simulink model "Lab0_actual"  (R2024b)
settings: Solver=ode5  StartTime=0.0  StopTime=20  FixedStep=1e-03  RelTol=1e-3
undefined symbols (not defined in the file): degs2rpm, delta_i, DiscIntNeverNeededParam, gbox, Kd, Ki, Kp, mot, National_Instruments, PCI, sens, TL, wc, wc2
libraries: simulink x9, sldrtlib x3
settings Model: SimulationMode=external  ExtModeTrigDuration=45001  Creator=lenovo  LastModifiedBy=aboulenien
settings DataIOCC: ReturnWorkspaceOutputs=off
settings HardwareCC: ProdBitPerLong=64  ProdHWDeviceType=Intel->x86-64 (Linux 64)
settings RTWCC: Description=Simulink Desktop Real-Time  SystemTargetFile=sldrt.tlc  TemplateMakefile=sldrt.tmf  RTWCompilerOptimization=on
settings CodeAppCC: MaxIdLength=95
settings SimulinkDesktopRealTimeCC: TargetLibSuffix=_sldrt.a  TargetPreCompLibLocation=C:\Program Files\MATLAB\R2024b\toolbox\sldrt\lib\win64  ParMdlRefBuildCompliant=on

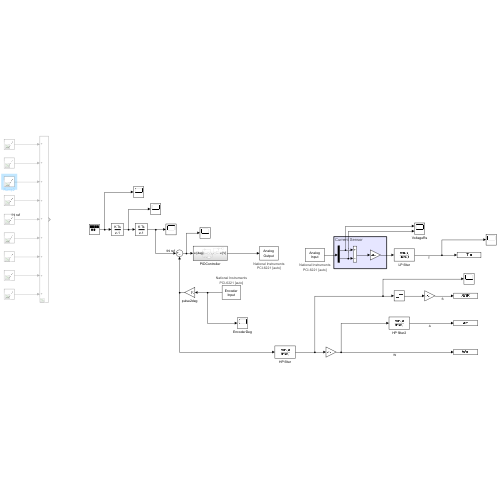
[thumbnail: Simulink's stored preview of the top-level diagram]
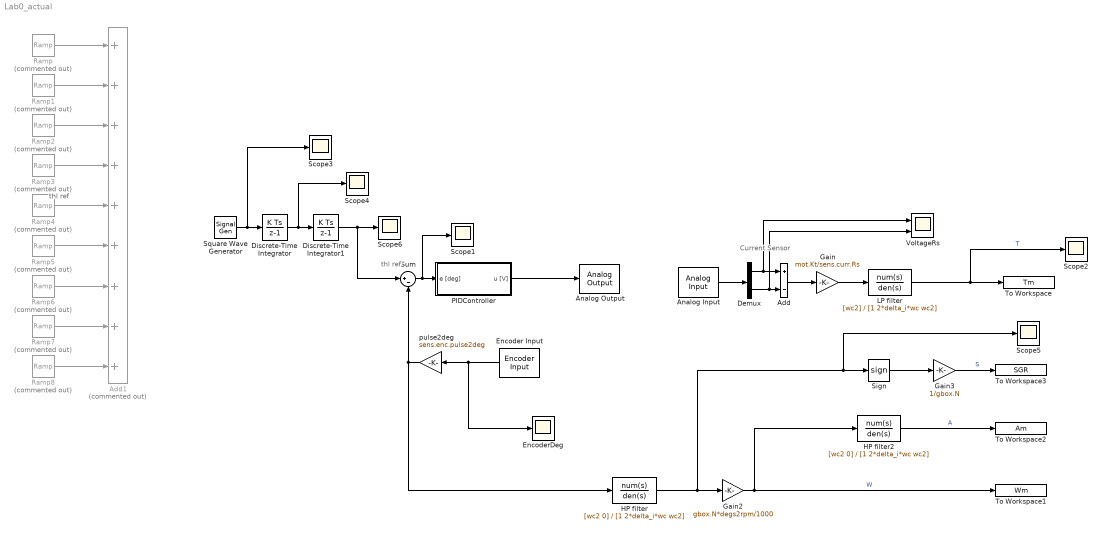
== system Lab0_actual ==
  note: Current Sensor
  note: thl ref
  note: thl ref
  Add : Sum  Inputs=+-
  Add1 : Sum  Commented=on  Inputs=+++++++++
  Analog Input : sldrtlib/Analog Input  SampleTime=-1  MaxMissedTicks=10  ShowMissedTicks=off  YieldWhenWaiting=off  DrvName=National_Instruments/PCI-6221  DrvAddress=4294967295  DrvOptions=[0 0 0 2 0]  Channels=[1,2]  RangeMode=1  VoltRange=1  DataType=1
      settings: AttributesFormatString=National Instruments\nPCI-6221 [auto]
  Analog Output : sldrtlib/Analog Output  SampleTime=-1  MaxMissedTicks=10  ShowMissedTicks=off  YieldWhenWaiting=off  DrvName=National_Instruments/PCI-6221  DrvAddress=4294967295  DrvOptions=[0 0 0 2 0]  Channels=1  RangeMode=1  VoltRange=1  InitialValue=0  FinalValue=0
      settings: AttributesFormatString=National Instruments\nPCI-6221 [auto]
  Demux : Demux  Outputs=2
  Discrete-Time Integrator : DiscreteIntegrator  SampleTime=-1  ICPrevOutput=DiscIntNeverNeededParam  ICPrevScaledInput=DiscIntNeverNeededParam
  Discrete-Time Integrator1 : DiscreteIntegrator  SampleTime=-1  ICPrevOutput=DiscIntNeverNeededParam  ICPrevScaledInput=DiscIntNeverNeededParam
  Encoder Input : sldrtlib/Encoder Input  SampleTime=-1  MaxMissedTicks=10  ShowMissedTicks=off  YieldWhenWaiting=off  DrvName=National_Instruments/PCI-6221  DrvAddress=4294967295  DrvOptions=[0 0 0 2 0]  Channels=1  QuadMode=3  IndexPulse=1  InputFilter=Inf  DataType=1
      settings: AttributesFormatString=National Instruments\nPCI-6221 [auto]
  EncoderDeg : Scope
  Gain : Gain  Gain=mot.Kt/sens.curr.Rs
  Gain2 : Gain  Gain=gbox.N*degs2rpm/1000
  Gain3 : Gain  Gain=1/gbox.N
  HP filter : TransferFcn  Numerator=[wc2 0]  Denominator=[1 2*delta_i*wc wc2]
  HP filter2 : TransferFcn  Numerator=[wc2 0]  Denominator=[1 2*delta_i*wc wc2]
  LP filter : TransferFcn  Numerator=[wc2]  Denominator=[1 2*delta_i*wc wc2]
  PIDController : Subsystem
  Ramp : simulink/Sources/Ramp  Commented=on  slope=300  start=0  InitialOutput=0
  Ramp1 : simulink/Sources/Ramp  Commented=on  slope=300  start=5  InitialOutput=0
  Ramp2 : simulink/Sources/Ramp  Commented=on  slope=300  start=10  InitialOutput=0
  Ramp3 : simulink/Sources/Ramp  Commented=on  slope=300  start=15  InitialOutput=0
  Ramp4 : simulink/Sources/Ramp  Commented=on  slope=300  start=20  InitialOutput=0
  Ramp5 : simulink/Sources/Ramp  Commented=on  slope=300  start=25  InitialOutput=0
  Ramp6 : simulink/Sources/Ramp  Commented=on  slope=300  start=30  InitialOutput=0
  Ramp7 : simulink/Sources/Ramp  Commented=on  slope=300  start=35  InitialOutput=0
  Ramp8 : simulink/Sources/Ramp  Commented=on  slope=300  start=40  InitialOutput=0
  Scope{1..6} (6 alike) : Scope
  Sign : Signum
  Square Wave Generator : SignalGenerator  WaveForm=square  Amplitude=2700  Frequency=0.5
  Sum : Sum  Inputs=|+-
  To Workspace : ToWorkspace  VariableName=Tm  SaveFormat=Structure With Time  SampleTime=0.1
  To Workspace1 : ToWorkspace  VariableName=Wm  SaveFormat=Structure With Time  SampleTime=0.1
  To Workspace2 : ToWorkspace  VariableName=Am  SaveFormat=Structure With Time  SampleTime=0.1
  To Workspace3 : ToWorkspace  VariableName=SGR  SaveFormat=Structure With Time  SampleTime=0.1
  VoltageRs : Scope  NumInputPorts=2
  pulse2deg : Gain  Gain=sens.enc.pulse2deg
  wires:
  Encoder Input/1 -> EncoderDeg/1, pulse2deg/1
  Sum/1 -> PIDController/1(e [deg]), Scope1/1
  pulse2deg/1 -> Sum/2, HP filter/1
  Demux/2 -> VoltageRs/2, Add/2
  Analog Input/1 -> Demux/1
  Demux/1 -> VoltageRs/1, Add/1
  Ramp2/1 -> Add1/3
  Ramp1/1 -> Add1/2
  Ramp4/1 -> Add1/5
  Ramp3/1 -> Add1/4
  Ramp5/1 -> Add1/6
  Ramp6/1 -> Add1/7
  Ramp8/1 -> Add1/9
  Ramp7/1 -> Add1/8
  Ramp/1 -> Add1/1
  HP filter/1 -> Scope5/1, Sign/1, Gain2/1
  Sign/1 -> Gain3/1
  Gain2/1 -> HP filter2/1, To Workspace1/1  "W"
  HP filter2/1 -> To Workspace2/1  "A"
  Gain3/1 -> To Workspace3/1  "S"
  Gain/1 -> LP filter/1
  LP filter/1 -> Scope2/1, To Workspace/1  "T"
  Add/1 -> Gain/1
  PIDController/1(u [V]) -> Analog Output/1
  Square Wave Generator/1 -> Discrete-Time Integrator/1, Scope3/1
  Discrete-Time Integrator/1 -> Scope4/1, Discrete-Time Integrator1/1
  Discrete-Time Integrator1/1 -> Sum/1, Scope6/1

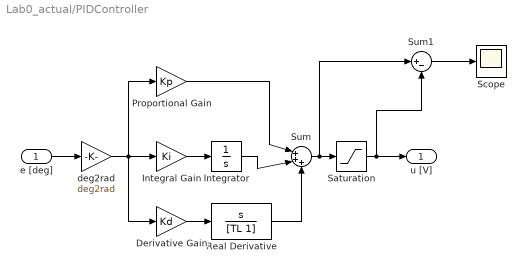
== system Lab0_actual/PIDController ==
  e [deg] : Inport
  Derivative Gain : Gain  Gain=Kd
  Integral Gain : Gain  Gain=Ki
  Integrator : Integrator
  Proportional Gain : Gain  Gain=Kp
  Real Derivative : TransferFcn  Numerator=[1 0]  Denominator=[TL 1]
  Saturation : Saturate  UpperLimit=12  LowerLimit=-12
  Scope : Scope
  Sum : Sum  Inputs=|+++
  Sum1 : Sum  Inputs=|+-
  deg2rad : Gain  Gain=deg2rad
  u [V] : Outport
  wires:
  Saturation/1 -> Sum1/2, u [V]/1
  Sum/1 -> Sum1/1, Saturation/1
  Real Derivative/1 -> Sum/3
  Sum1/1 -> Scope/1
  Integral Gain/1 -> Integrator/1
  deg2rad/1 -> Derivative Gain/1, Proportional Gain/1, Integral Gain/1
  Integrator/1 -> Sum/2
  e [deg]/1 -> deg2rad/1
  Proportional Gain/1 -> Sum/1
  Derivative Gain/1 -> Real Derivative/1
